simulink model "supplemental_network"  (R2023b)
settings: Solver=ode3  StartTime=0.0  StopTime=sup_cfg.stop  FixedStep=sup_cfg.electricalStep  RelTol=1e-6
InitFcn:
  | Rf=0.05;Lf=2e-3;Cf=50e-6;fn=50;w0=2*fn*pi;
  | UB=3e3;SB=1e6;IB=SB/(sqrt(3)*UB);
  | Xf=Lf*w0;Z=sqrt((Rf^2+Xf^2));
  | J=3;D=2e4/w0*0;kf=0.9e4/w0;
  | K=230*380/Xf;
  | P=10;I=12e3;
  | Jw=8e4;
  | Pi=1;Pp=0;P2 =1000;
  | U5=30;
  | U7=15;
undefined symbols (not defined in the file): sup_cfg
libraries: slpidlib x5, spsThreePhaseSeriesRLCBranchLib x4, spsControlledVoltageSourceLib x4, spsControlledCurrentSourceLib x3, spsThreePhaseBreakerLib x3, spsabctodq0Lib x3, spsThreePhaseVIMeasurementLib x3, spsGroundLib x2, spsThreePhaseSeriesRLCLoadLib x2, spsUniversalBridgeLib x1, spsPWMGenerator2LevelLib x1, spsdq0toabcLib x1
settings Model: Creator=lenovo  LastModifiedBy=yangweilin
settings SolverCC: ZeroCrossAlgorithm=Adaptive  AlgebraicLoopSolver=TrustRegion
settings DataIOCC: SaveFormat=StructureWithTime  SignalLogging=off
settings OptimizationCC: DefaultParameterBehavior=Inlined  EnhancedBackFolding=on  PassReuseOutputArgsAs=Individual arguments  ZeroExternalMemoryAtStartup=off  ZeroInternalMemoryAtStartup=off  AccelVerboseBuild=on  OptimizeBlockOrder=speed  DifferentSizesBufferReuse=on  OptimizationCustomize=off  EfficientTunableParamExpr=on
settings DebuggingCC: IgnoredZcDiagnostic=none  ParameterTunabilityLossMsg=error  UnconnectedInputMsg=warning  UnconnectedOutputMsg=warning  UnconnectedLineMsg=warning  ArithmeticOperatorsInVariantConditions=warning
settings ModelReferenceCC: EnableRefExpFcnMdlSchedulingChecks=on
settings SFSimCC: MATLABDynamicMemAlloc=off  CustomCodeUndefinedFunction=UseInterfaceOnly
settings RTWCC: Description=Embedded Coder  SystemTargetFile=ert.tlc  TemplateMakefile=ert_default_tmf
settings CodeAppCC: ForceParamTrailComments=on  IgnoreCustomStorageClasses=off  OperatorAnnotations=on  SimulinkDataObjDesc=on  SFDataObjDesc=on  InsertBlockDesc=on
settings ERTTargetCC: TargetLangStandard=C99 (ISO)  GenerateSampleERTMain=on  InlinedParameterPlacement=NonHierarchical  ERTCustomFileTemplate=example_file_process.tlc

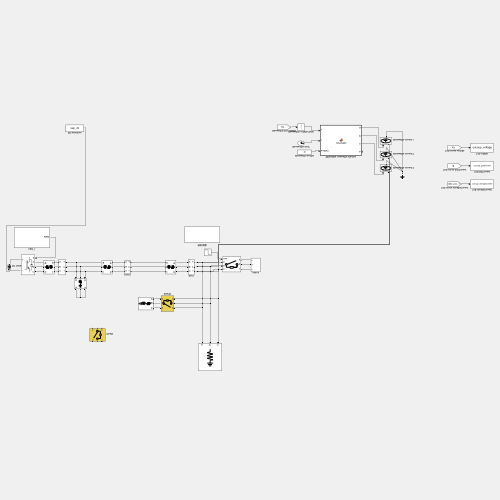
[thumbnail: Simulink's stored preview of the top-level diagram]
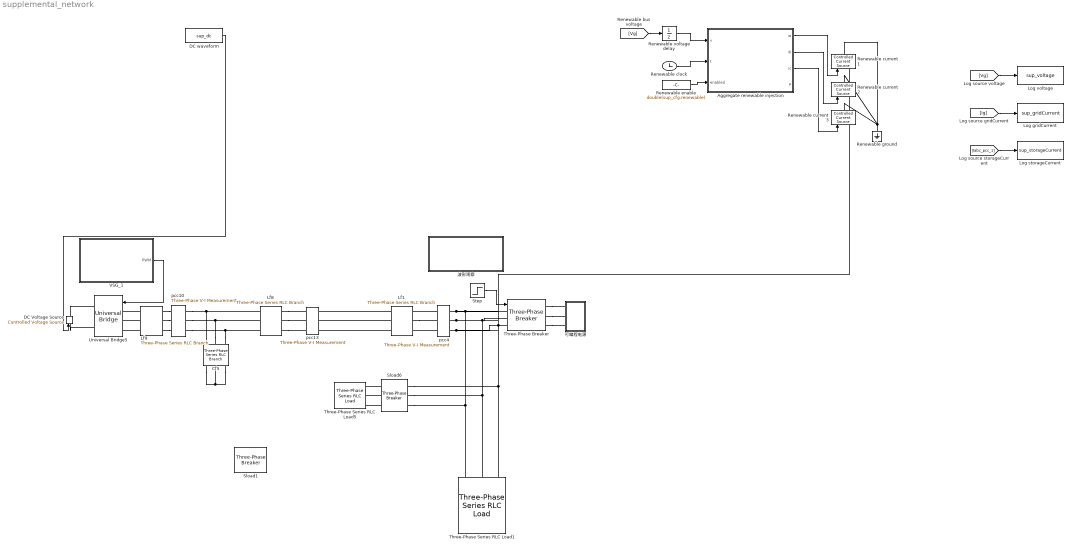
== system supplemental_network ==
  " Lf1" : spsThreePhaseSeriesRLCBranchLib/Three-Phase Series RLC Branch  LConnTagsString=A|B|C  RConnTagsString=A|B|C  BranchType=RL  Resistance=0.1  Inductance=0.0002  Capacitance=0  Measurements=None
  " Lf8" : spsThreePhaseSeriesRLCBranchLib/Three-Phase Series RLC Branch  LConnTagsString=A|B|C  RConnTagsString=A|B|C  BranchType=RL  Resistance=0.02  Inductance=0.004  Capacitance=0  Measurements=None
  " Lf9" : spsThreePhaseSeriesRLCBranchLib/Three-Phase Series RLC Branch  LConnTagsString=A|B|C  RConnTagsString=A|B|C  BranchType=RL  Resistance=0.1  Inductance=0.005  Capacitance=0  Measurements=None
  Aggregate renewable injection : MATLAB Function  TreatAsAtomicUnit=on
  Cf5 : spsThreePhaseSeriesRLCBranchLib/Three-Phase Series RLC Branch  LConnTagsString=A|B|C  RConnTagsString=A|B|C  BranchType=RC  Resistance=0.5  Inductance=4e-3  Capacitance=3e-5  Measurements=None
  DC Voltage Source : spsControlledVoltageSourceLib/Controlled Voltage Source  Initialize=on  Source_Type=DC  Amplitude=800  Phase=0  Frequency=0  Measurements=None
  DC waveform : FromWorkspace  VariableName=sup_dc  Interpolate=off  OutputAfterFinalValue=Holding final value
  Log gridCurrent : ToWorkspace  VariableName=sup_gridCurrent  SaveFormat=Structure With Time  SampleTime=sup_cfg.Ts
  Log storageCurrent : ToWorkspace  VariableName=sup_storageCurrent  SaveFormat=Structure With Time  SampleTime=sup_cfg.Ts
  Log voltage : ToWorkspace  VariableName=sup_voltage  SaveFormat=Structure With Time  SampleTime=sup_cfg.Ts
  Renewable clock : Clock
  Renewable current 1 : spsControlledCurrentSourceLib/Controlled Current Source  Initialize=on  Source_Type=DC  Amplitude=0  Phase=0  Frequency=0  Measurements=None
  Renewable current 2 : spsControlledCurrentSourceLib/Controlled Current Source  Initialize=on  Source_Type=DC  Amplitude=0  Phase=0  Frequency=0  Measurements=None
  Renewable current 3 : spsControlledCurrentSourceLib/Controlled Current Source  Initialize=on  Source_Type=DC  Amplitude=0  Phase=0  Frequency=0  Measurements=None
  Renewable enable : Constant  Value=double(sup_cfg.renewable)
  Renewable ground : spsGroundLib/Ground  LConnTagsString=a
  Renewable voltage delay : UnitDelay  InitialCondition=[0;0;0]  SampleTime=sup_cfg.electricalStep  HasFrameUpgradeWarning=on
  Sload1 : spsThreePhaseBreakerLib/Three-Phase Breaker  InitialState=open  SwitchA=on  SwitchB=on  SwitchC=on  SwitchTimes=[1.0]  External=off  BreakerResistance=0.0001  SnubberResistance=1e6  SnubberCapacitance=inf  Measurements=None
  Sload6 : spsThreePhaseBreakerLib/Three-Phase Breaker  InitialState=open  SwitchA=on  SwitchB=on  SwitchC=on  SwitchTimes=[1.2]  External=off  BreakerResistance=0.0001  SnubberResistance=1e6  SnubberCapacitance=inf  Measurements=None
  Step : Step  Before=1  After=0  SampleTime=0
  Three-Phase Series RLC Load1 : spsThreePhaseSeriesRLCLoadLib/Three-Phase Series RLC Load  LConnTagsString=A|B|C  Configuration=Y (grounded)  NominalVoltage=380  Vabc=[1e3 1e3 1e3]  Vabcp=[1e3 1e3 1e3]  NominalFrequency=50  UnbalancedPower=off  ActivePower=15e3  InductivePower=0  CapacitivePower=0  Pabc=[10e3 9e3 11e3]  QLabc=[100 90 110]  QCabc=[100 90 110]  Pabcp=[10e3 9e3 11e3]  QLabcp=[100 90 110]  QCabcp=[100 90 110]  Measurements=None  LoadType=constant Z
  Three-Phase Series RLC Load5 : spsThreePhaseSeriesRLCLoadLib/Three-Phase Series RLC Load  LConnTagsString=A|B|C  Configuration=Y (grounded)  NominalVoltage=380  Vabc=[1e3 1e3 1e3]  Vabcp=[1e3 1e3 1e3]  NominalFrequency=50  UnbalancedPower=off  ActivePower=15e3  InductivePower=6e3  CapacitivePower=0  Pabc=[10e3 9e3 11e3]  QLabc=[100 90 110]  QCabc=[100 90 110]  Pabcp=[10e3 9e3 11e3]  QLabcp=[100 90 110]  QCabcp=[100 90 110]  Measurements=None  LoadType=constant Z
  Three-Phase Breaker : spsThreePhaseBreakerLib/Three-Phase Breaker  InitialState=open  SwitchA=on  SwitchB=on  SwitchC=on  SwitchTimes="[1/60  5/60]"  External=on  BreakerResistance=0.01  SnubberResistance=1e6  SnubberCapacitance=inf  Measurements=None
  Universal Bridge5 : spsUniversalBridgeLib/Universal Bridge  Arms=3  SnubberResistance=1e5  SnubberCapacitance=inf  Device=IGBT / Diodes  Ron=1e-5  Lon=0  ForwardVoltages=[0.05 0.05]  ForwardVoltage=0  GTOparameters=[ 10e-6 , 20e-6 ]  IGBTparameters=[ 1e-6 , 2e-6 ]  Measurements=None  Measurements_2=None  converterType=Rectifier
  VSG_1 : Subsystem
  pcc10 : spsThreePhaseVIMeasurementLib/Three-Phase V-I Measurement  VoltageMeasurement=phase-to-ground  SetLabelV=on  LabelV=Vo_1  Vpu=off  VpuLL=off  CurrentMeasurement=yes  SetLabelI=on  LabelI=IL_1  Ipu=off  Pbase=1e6  Vbase=6.6e3/sqrt(3)  OutputType=Magnitude  PhasorSimulation=off  PSBequivalent=0
  pcc13 : spsThreePhaseVIMeasurementLib/Three-Phase V-I Measurement  VoltageMeasurement=phase-to-ground  SetLabelV=on  LabelV=Vabc_pcc_1  Vpu=off  VpuLL=off  CurrentMeasurement=yes  SetLabelI=on  LabelI=Iabc_pcc_1  Ipu=off  Pbase=1e6  Vbase=6.6e3/sqrt(3)  OutputType=Magnitude  PhasorSimulation=off  PSBequivalent=0
  pcc4 : spsThreePhaseVIMeasurementLib/Three-Phase V-I Measurement  VoltageMeasurement=phase-to-ground  SetLabelV=on  LabelV=Vg  Vpu=off  VpuLL=off  CurrentMeasurement=yes  SetLabelI=on  LabelI=Ig  Ipu=off  Pbase=1e6  Vbase=6.6e3/sqrt(3)  OutputType=Magnitude  PhasorSimulation=off  PSBequivalent=0
  可编程电源 : Subsystem
  波形观察 : Subsystem
  wires:
  VSG_1/1(PWM) -> Universal Bridge5/1
  Step/1 -> Three-Phase Breaker/1
  DC waveform/1 -> DC Voltage Source/1
  [Vg] -> Renewable voltage delay/1
  Renewable voltage delay/1 -> Aggregate renewable injection/1(v)
  Renewable clock/1 -> Aggregate renewable injection/2(t)
  Renewable enable/1 -> Aggregate renewable injection/3(enabled)
  Aggregate renewable injection/1(ia) -> Renewable current 1/1
  Aggregate renewable injection/2(ib) -> Renewable current 2/1
  Aggregate renewable injection/3(ic) -> Renewable current 3/1
  [Vg] -> Log voltage/1
  [Ig] -> Log gridCurrent/1
  [Iabc_pcc_1] -> Log storageCurrent/1
  connections:
  Cf5/RConn2 -- Cf5/RConn3 -- Cf5/RConn1
  " Lf9"/LConn3 -- Universal Bridge5/LConn3
  " Lf9"/LConn1 -- Universal Bridge5/LConn1
  " Lf9"/LConn2 -- Universal Bridge5/LConn2
  " Lf8"/RConn1 -- pcc10/RConn1 -- Cf5/LConn1
  Cf5/LConn3 -- pcc10/RConn3 -- " Lf8"/RConn3
  Cf5/LConn2 -- pcc10/RConn2 -- " Lf8"/RConn2
  " Lf1"/LConn2 -- pcc4/LConn2
  pcc4/LConn3 -- " Lf1"/LConn3
  pcc4/LConn1 -- " Lf1"/LConn1
  " Lf1"/RConn1 -- pcc13/RConn1
  " Lf1"/RConn2 -- pcc13/RConn2
  " Lf1"/RConn3 -- pcc13/RConn3
  " Lf8"/LConn1 -- pcc13/LConn1
  " Lf8"/LConn2 -- pcc13/LConn2
  " Lf8"/LConn3 -- pcc13/LConn3
  DC Voltage Source/RConn1 -- Universal Bridge5/RConn1
  DC Voltage Source/LConn1 -- Universal Bridge5/RConn2
  " Lf9"/RConn1 -- pcc10/LConn1
  " Lf9"/RConn2 -- pcc10/LConn2
  " Lf9"/RConn3 -- pcc10/LConn3
  Three-Phase Breaker/RConn1 -- 可编程电源/RConn1
  Three-Phase Breaker/RConn2 -- 可编程电源/RConn2
  Three-Phase Breaker/RConn3 -- 可编程电源/RConn3
  Sload6/LConn3 -- Three-Phase Series RLC Load5/LConn1
  Sload6/LConn2 -- Three-Phase Series RLC Load5/LConn2
  Sload6/LConn1 -- Three-Phase Series RLC Load5/LConn3
  Three-Phase Breaker/LConn1 -- Three-Phase Series RLC Load1/LConn1 -- Sload6/RConn1 -- pcc4/RConn1 -- Renewable current 1/LConn1
  pcc4/RConn2 -- Renewable current 2/LConn1 -- Three-Phase Series RLC Load1/LConn2 -- Sload6/RConn2 -- Three-Phase Breaker/LConn2
  Three-Phase Breaker/LConn3 -- Sload6/RConn3 -- Three-Phase Series RLC Load1/LConn3 -- pcc4/RConn3 -- Renewable current 3/LConn1
  Renewable current 1/RConn1 -- Renewable current 2/RConn1 -- Renewable ground/LConn1 -- Renewable current 3/RConn1

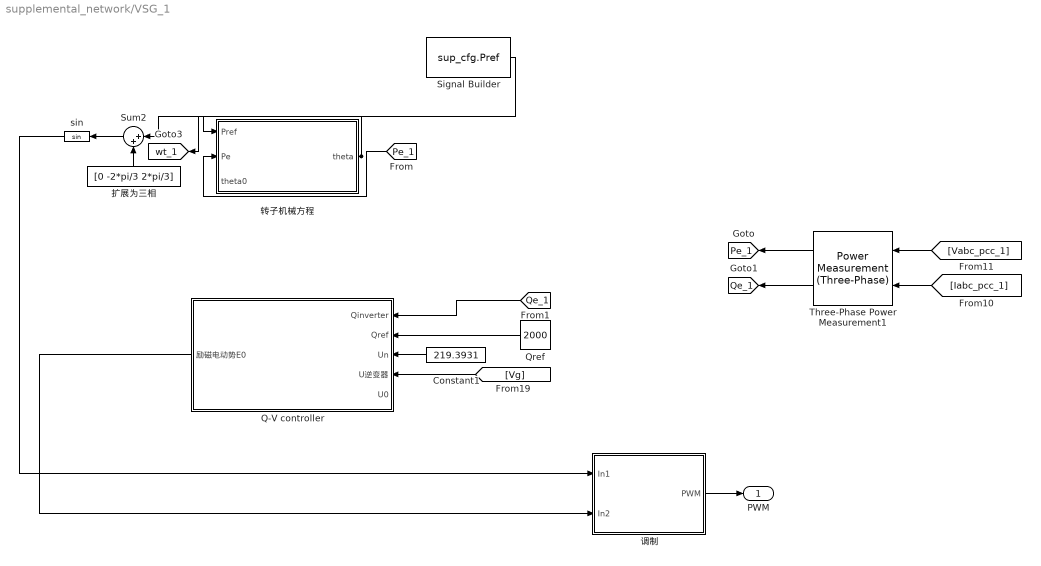
== system supplemental_network/VSG_1 ==
  " 调制" : Subsystem
  Constant1 : Constant  Value=219.3931
  Q-V controller : Subsystem
  Qref : Constant  Value=2000
  Signal Builder : Constant  Value=sup_cfg.Pref
  Sum2 : Sum  Inputs=|++
  Three-Phase Power Measurement1 : eePowerMeasurement/Power Measurement (Three-Phase)  LabelModeActiveChoice=Continuous  F=50  K=[1]  Seq=Positive  Ts=0
  sin : Trigonometry
  扩展为三相 : Constant  Value=[0 -2*pi/3 2*pi/3]
  转子机械方程 : Subsystem
  PWM : Outport
  tag scope: Pe_1=global, Qe_1=global, wt_1=global
  wires:
  扩展为三相/1 -> Sum2/2
  Three-Phase Power Measurement1/1 -> [Pe_1]
  [Iabc_pcc_1] -> Three-Phase Power Measurement1/2
  Qref/1 -> Q-V controller/2(Qref)
  [Vg] -> Q-V controller/4(U逆变器)
  [Vabc_pcc_1] -> Three-Phase Power Measurement1/1
  Three-Phase Power Measurement1/2 -> [Qe_1]
  Constant1/1 -> Q-V controller/3(Un)
  Sum2/1 -> sin/1
  sin/1 -> " 调制"/1(In1)
  Q-V controller/1(励磁电动势E0) -> " 调制"/2(In2)
  " 调制"/1(PWM) -> PWM/1
  [Qe_1] -> Q-V controller/1(Qinverter)
  [Pe_1] -> 转子机械方程/2(Pe)
  转子机械方程/1(theta) -> Sum2/1, [wt_1]
  Signal Builder/1 -> 转子机械方程/1(Pref)

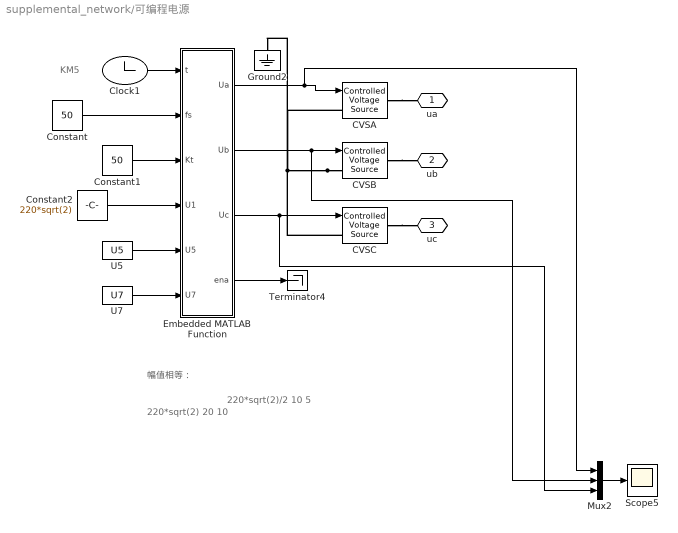
== system supplemental_network/可编程电源 ==
  note: KM5
  note: 幅值相等：
  note: 220*sqrt(2)
      | 20
      | 10
  note: 220*sqrt(2)/2
      | 10
      | 5
  CVSA : spsControlledVoltageSourceLib/Controlled Voltage Source  Initialize=on  Source_Type=AC  Amplitude=0  Phase=0  Frequency=0  Measurements=None
  CVSB : spsControlledVoltageSourceLib/Controlled Voltage Source  Initialize=on  Source_Type=AC  Amplitude=0  Phase=0  Frequency=0  Measurements=None
  CVSC : spsControlledVoltageSourceLib/Controlled Voltage Source  Initialize=on  Source_Type=AC  Amplitude=0  Phase=0  Frequency=0  Measurements=None
  Clock1 : Clock
  Constant : Constant  Value=50
  Constant1 : Constant  Value=50
  Constant2 : Constant  Value=220*sqrt(2)
  Embedded MATLAB Function : MATLAB Function  TreatAsAtomicUnit=on
  Ground2 : spsGroundLib/Ground  LConnTagsString=a
  Mux2 : Mux  Inputs=3
  Scope5 : Scope
  Terminator4 : Terminator
  U5 : Constant  Value=U5
  U7 : Constant  Value=U7
  ua : PMIOPort  Side=Right
  ub : PMIOPort  Port=2  Side=Right
  uc : PMIOPort  Port=3  Side=Right
  wires:
  Clock1/1 -> Embedded MATLAB Function/1(t)
  U5/1 -> Embedded MATLAB Function/5(U5)
  Embedded MATLAB Function/3(Uc) -> Mux2/3, CVSC/1
  U7/1 -> Embedded MATLAB Function/6(U7)
  Embedded MATLAB Function/4(ena) -> Terminator4/1
  Constant1/1 -> Embedded MATLAB Function/3(Kt)
  Constant/1 -> Embedded MATLAB Function/2(fs)
  Embedded MATLAB Function/2(Ub) -> Mux2/2, CVSB/1
  Mux2/1 -> Scope5/1
  Embedded MATLAB Function/1(Ua) -> Mux2/1, CVSA/1
  Constant2/1 -> Embedded MATLAB Function/4(U1)
  connections:
  CVSC/RConn1 -- uc/RConn1
  CVSB/RConn1 -- ub/RConn1
  CVSA/RConn1 -- ua/RConn1
  CVSB/LConn1 -- Ground2/LConn1 -- CVSA/LConn1 -- CVSC/LConn1

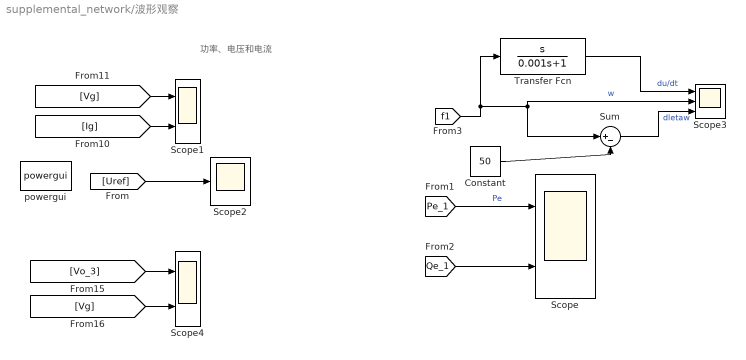
== system supplemental_network/波形观察 ==
  note: 功率、电压和电流
  Constant : Constant  Value=50
  Scope : Scope  NumInputPorts=2
  Scope1 : Scope  NumInputPorts=2
  Scope2 : Scope
  Scope3 : Scope  NumInputPorts=3
  Scope4 : Scope  NumInputPorts=2
  Sum : Sum  Inputs=|+-
  Transfer Fcn : TransferFcn  Numerator=[1 0]  Denominator=[0.001 1]
  powergui : spspowerguiLib/powergui  Priority=1  SimulationMode=Discrete  SampleTime=sup_cfg.electricalStep  frequency=60  Iterations=50  frequencyindice=0  Pbase=100e6  ErrMax=1e-4  UnitsV=kV  UnitsW=MW  buscounter=0  FunctionMessages=off  echomessages=off  EnableUseOfTLC=off  CurrentSourceSwitches=off  DisableSnubberDevices=off  DisableRonSwitches=off  DisableVfSwitches=off  DisplayEquations=off  AutomaticDiscreteSolvers=off  SolverType=Tustin/Backward Euler (TBE)  Interpol=off  ExternalGateDelay=off  methode=off  Ts=100  x0status=blocks  SPID=on  SwTol=0  HookPort=off  NonlinearTolerance=1e-4  nMaxIteration=100  ContinueOnMaxIteration=off  RestoreLinks=warning  ResistiveCurrentMeasurement=off  Frange=[0:2:500]  Ylog=off  Xlog=on  ShowGrid=off  save=off  variable=ZData  structure=logsout  ZoomFFT=off  StartTime=0.5  cycles=10  DisplayStyle=1  fundamental=50  FreqAxis=off  MaxFrequency=1000  frequencyindicesteady=1  RmsSteady=1  display=off
  wires:
  [Vg] -> Scope1/1
  [Qe_1] -> Scope/2
  [Pe_1] -> Scope/1  "Pe"
  [Ig] -> Scope1/2
  [Uref] -> Scope2/1
  [f1] -> Sum/1, Scope3/2, Transfer Fcn/1  "w"
  [Vo_3] -> Scope4/1
  [Vg] -> Scope4/2
  Transfer Fcn/1 -> Scope3/1  "du/dt"
  Constant/1 -> Sum/2
  Sum/1 -> Scope3/3  "dletaw"

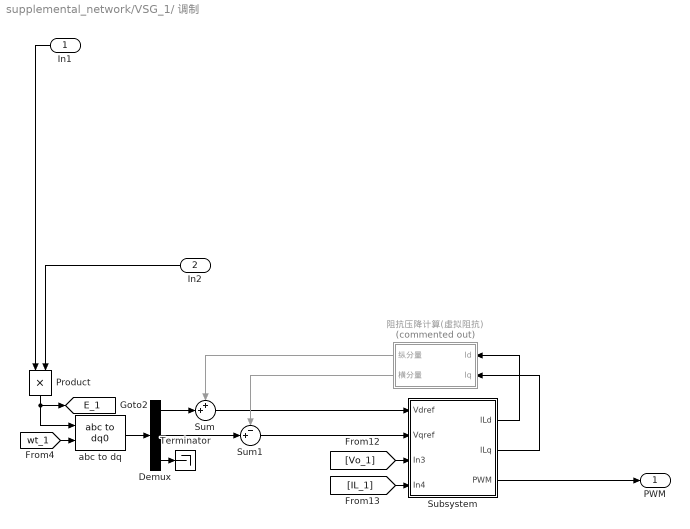
== system supplemental_network/VSG_1/ 调制 ==
  In1 : Inport
  In2 : Inport  Port=2
  Demux : Demux  Outputs=3
  Product : Product
  Subsystem : Subsystem
  Sum : Sum  Inputs=++|
  Sum1 : Sum  Inputs=-+|
  Terminator : Terminator
  abc to dq : spsabctodq0Lib/abc to dq0  Alignment=90 degrees behind phase A axis
  阻抗压降计算(虚拟阻抗) : Subsystem  Commented=on
  PWM : Outport
  tag scope: E_1=global
  wires:
  [Vo_1] -> Subsystem/3(In3)
  Demux/2 -> Sum1/2
  Sum/1 -> Subsystem/1(Vdref)
  [IL_1] -> Subsystem/4(In4)
  abc to dq/1 -> Demux/1
  Subsystem/1(ILd) -> 阻抗压降计算(虚拟阻抗)/1(Id)
  Demux/1 -> Sum/2
  阻抗压降计算(虚拟阻抗)/1(纵分量) -> Sum/1
  Demux/3 -> Terminator/1
  Sum1/1 -> Subsystem/2(Vqref)
  Product/1 -> [E_1], abc to dq/1
  Subsystem/2(ILq) -> 阻抗压降计算(虚拟阻抗)/2(Iq)
  阻抗压降计算(虚拟阻抗)/2(横分量) -> Sum1/1
  Subsystem/3(PWM) -> PWM/1
  [wt_1] -> abc to dq/2
  In1/1 -> Product/1
  In2/1 -> Product/2

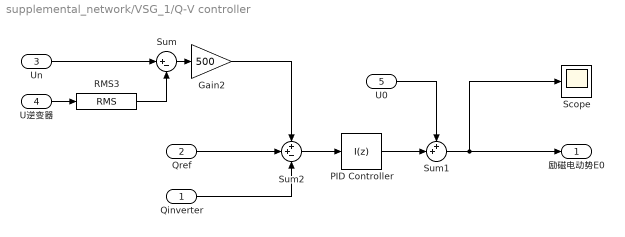
== system supplemental_network/VSG_1/Q-V controller ==
  Qinverter : Inport
  Qref : Inport  Port=2
  Un : Inport  Port=3
  U逆变器 : Inport  Port=4
  U0 : Inport  Port=5
  Gain2 : Gain  Gain=500
  PID Controller : slpidlib/PID Controller  Controller=I  Form=Parallel  TimeDomain=Discrete-time  UseExternalTs=off  SampleTime=-1  IntegratorMethod=Forward Euler  FilterMethod=Forward Euler  ControllerParametersSource=internal  P=0.0000001  I=1.1547e-5*5  UseKiTs=off  D=0  N=100  UseFilter=on  TunerSelectOption=Transfer Function Based (PID Tuner App)  InitialConditionSource=internal  InitialConditionForIntegrator=0  InitialConditionForFilter=0  DifferentiatorICPrevScaledInput=0  ExternalReset=none  TrackingMode=off  Kt=1  LimitOutput=off  SatLimitsSource=internal  UpperSaturationLimit=inf  LowerSaturationLimit=-inf  LinearizeAsGain=on  AntiWindupMode=none  Kb=1  LimitIntegrator=off  UpperIntegratorSaturationLimit=inf  LowerIntegratorSaturationLimit=-inf  POutMin=[]  POutMax=[]  IOutMin=[]  IOutMax=[]  DOutMin=[]  DOutMax=[]  NOutMin=[]  NOutMax=[]  SumOutMin=[]  SumOutMax=[]  SaturationOutMin=[]  SaturationOutMax=[]  PParamMin=[]  PParamMax=[]  IParamMin=[]  IParamMax=[]  DParamMin=[]  DParamMax=[]  NParamMin=[]  NParamMax=[]  KbParamMin=[]  KbParamMax=[]  KtParamMin=[]  KtParamMax=[]  KbOutMin=[]  KbOutMax=[]  KtOutMin=[]  KtOutMax=[]  IntegratorOutMin=[]  IntegratorOutMax=[]  FilterOutMin=[]  FilterOutMax=[]  SumI1OutMin=[]  SumI1OutMax=[]  SumI2OutMin=[]  SumI2OutMax=[]  SumI3OutMin=[]  SumI3OutMax=[]  SumI4OutMin=[]  SumI4OutMax=[]  SumDOutMin=[]  SumDOutMax=[]  DifferentiatorOutMin=[]  DifferentiatorOutMax=[]  FilterDiffOutCoefMin=[]  FilterDiffOutCoefMax=[]  ReciprocalOutMin=[]  ReciprocalOutMax=[]  SumDenOutMin=[]  SumDenOutMax=[]  SumNumOutMin=[]  SumNumOutMax=[]  DivideOutMin=[]  DivideOutMax=[]  UdiffTsProdOutMin=[]  UdiffTsProdOutMax=[]  NTsProdOutMin=[]  NTsProdOutMax=[]  UintegralTsProdOutMin=[]  UintegralTsProdOutMax=[]  UngainTsProdOutMin=[]  UngainTsProdOutMax=[]  ClampingZeroOutDataTypeStr=Inherit: Inherit via back propagation  ClampingZeroOutMin=[]  ClampingZeroOutMax=[]  FilterDenConstantOutDataTypeStr=Inherit: Inherit via back propagation  FilterDenConstantOutMin=[]  FilterDenConstantOutMax=[]  PCopyOutDataTypeStr=Inherit: Inherit via back propagation  PCopyOutMin=[]  PCopyOutMax=[]  NCopyOutDataTypeStr=Inherit: Inherit via back propagation  NCopyOutMin=[]  NCopyOutMax=[]  IntegratorContinuousStateAttributes=''  IntegratorStateMustResolveToSignalObject=off  IntegratorRTWStateStorageClass=Auto  FilterContinuousStateAttributes=''  FilterStateMustResolveToSignalObject=off  FilterRTWStateStorageClass=Auto  ParallelPVariant=Disabled  IdealPVariant=Disabled  IVariant=InternalParameters  DVariant=Disabled  IntegratorVariant=Discrete  SatVariant=Disabled  AWVariant=Passthrough  PCopyVariant=Disabled  TRVariant=Disabled  FdbkBlocksVariant=Forward  IdealPFdbkVariant=Disabled  SatFdbkVariant=Disabled  DerivativeFilterVariant=Disabled  NVariant=Disabled  NCopyVariant=Disabled_SignalSpec  FilterICVariant=Disabled  IntegratorICVariant=InternalICs  ExternalResetVariant=Disabled  TRSumVariant=Passthrough  SumFdbkVariant=Disabled  SumVariant=Passthrough_I  TsampFilterVariant=InternalTs  TsampNgainVariant=Passthrough  TsampIntegralVariant=Disabled_SignalSpec  ExternalSaturationOutDataTypeStr=Inherit: Same as second input
  RMS3 : dspstat3/RMS  run=off  directionMode=Each column  dimension=1  InputProcessing=Columns as channels (frame based)  reset_popup=None
  Scope : Scope
  Sum : Sum  Inputs=|+-
  Sum1 : Sum  Inputs=++|
  Sum2 : Sum  Inputs=++-
  励磁电动势E0 : Outport
  wires:
  Qinverter/1 -> Sum2/3
  Qref/1 -> Sum2/2
  Un/1 -> Sum/1
  U逆变器/1 -> RMS3/1
  Gain2/1 -> Sum2/1
  Sum/1 -> Gain2/1
  RMS3/1 -> Sum/2
  Sum2/1 -> PID Controller/1
  U0/1 -> Sum1/1
  Sum1/1 -> 励磁电动势E0/1, Scope/1
  PID Controller/1 -> Sum1/2

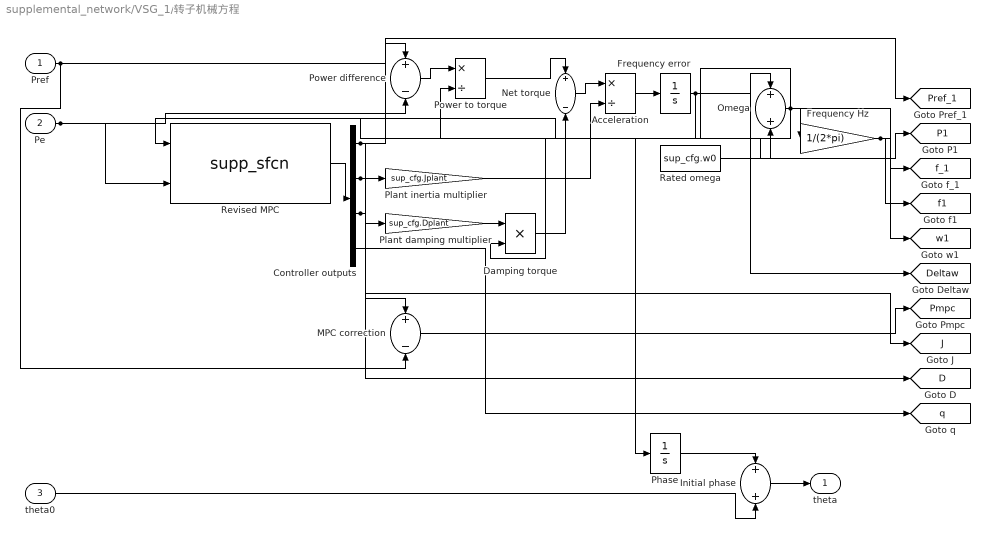
== system supplemental_network/VSG_1/转子机械方程 ==
  Pref : Inport
  Pe : Inport  Port=2
  theta0 : Inport  Port=3
  Acceleration : Product  Inputs=*/
  Controller outputs : Demux
  Damping torque : Product  Inputs=**
  Frequency Hz : Gain  Gain=1/(2*pi)
  Frequency error : Integrator
  Initial phase : Sum
  MPC correction : Sum  Inputs=+-
  Net torque : Sum  Inputs=+-
  Omega : Sum
  Phase : Integrator
  Plant damping multiplier : Gain  Gain=sup_cfg.Dplant
  Plant inertia multiplier : Gain  Gain=sup_cfg.Jplant
  Power difference : Sum  Inputs=+-
  Power to torque : Product  Inputs=*/
  Rated omega : Constant  Value=sup_cfg.w0
  Revised MPC : M-S-Function  FunctionName=supp_sfcn  Parameters=sup_cfg
  theta : Outport
  tag scope: D=global, Deltaw=global, J=global, P1=global, Pmpc=global, Pref_1=global, f1=global, f_1=global, q=global, w1=global
  wires:
  Pe/1 -> Revised MPC/2, Power difference/2, [P1]
  Omega/1 -> Revised MPC/1, Power to torque/2, Frequency Hz/1, Phase/1, [w1]
  Revised MPC/1 -> Controller outputs/1
  Controller outputs/1 -> Power difference/1, MPC correction/1
  Power difference/1 -> Power to torque/1
  Controller outputs/2 -> Plant inertia multiplier/1, [J]
  Controller outputs/3 -> Plant damping multiplier/1, [D]
  Plant damping multiplier/1 -> Damping torque/1
  Frequency error/1 -> Damping torque/2, Omega/1, [Deltaw]
  Power to torque/1 -> Net torque/1
  Damping torque/1 -> Net torque/2
  Net torque/1 -> Acceleration/1
  Plant inertia multiplier/1 -> Acceleration/2
  Acceleration/1 -> Frequency error/1
  Rated omega/1 -> Omega/2
  Phase/1 -> Initial phase/1
  theta0/1 -> Initial phase/2
  Initial phase/1 -> theta/1
  Pref/1 -> MPC correction/2, [Pref_1]
  Frequency Hz/1 -> [f_1], [f1]
  MPC correction/1 -> [Pmpc]
  Controller outputs/4 -> [q]

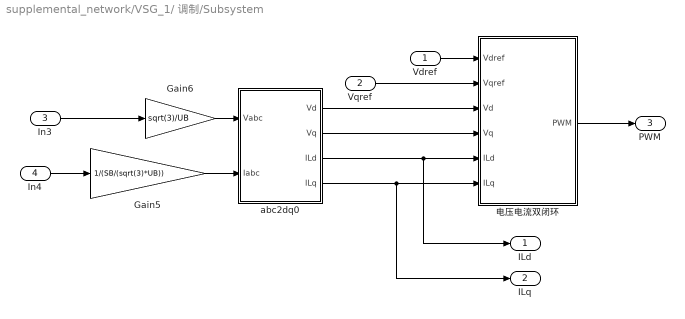
== system supplemental_network/VSG_1/ 调制/Subsystem ==
  Vdref : Inport
  Vqref : Inport  Port=2
  In3 : Inport  Port=3
  In4 : Inport  Port=4
  Gain5 : Gain  Gain=1/(SB/(sqrt(3)*UB))
  Gain6 : Gain  Gain=sqrt(3)/UB
  abc2dq0 : Subsystem
  电压电流双闭环 : Subsystem
  ILd : Outport
  ILq : Outport  Port=2
  PWM : Outport  Port=3
  wires:
  Vqref/1 -> 电压电流双闭环/2(Vqref)
  In4/1 -> Gain5/1
  abc2dq0/1(Vd) -> 电压电流双闭环/3(Vd)
  abc2dq0/2(Vq) -> 电压电流双闭环/4(Vq)
  abc2dq0/3(ILd) -> 电压电流双闭环/5(ILd), ILd/1
  Gain5/1 -> abc2dq0/2(Iabc)
  Gain6/1 -> abc2dq0/1(Vabc)
  abc2dq0/4(ILq) -> 电压电流双闭环/6(ILq), ILq/1
  电压电流双闭环/1(PWM) -> PWM/1
  Vdref/1 -> 电压电流双闭环/1(Vdref)
  In3/1 -> Gain6/1

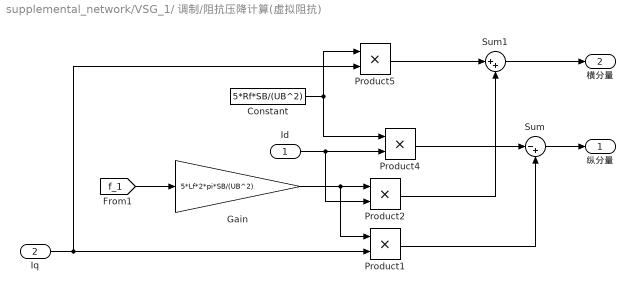
== system supplemental_network/VSG_1/ 调制/阻抗压降计算(虚拟阻抗) ==
  Id : Inport
  Iq : Inport  Port=2
  Constant : Constant  Value=5*Rf*SB/(UB^2)
  Gain : Gain  Gain=5*Lf*2*pi*SB/(UB^2)
  Product{1..2,4..5} (4 alike) : Product
  Sum : Sum  Inputs=|-+
  Sum1 : Sum  Inputs=|++
  纵分量 : Outport
  横分量 : Outport  Port=2
  wires:
  Product2/1 -> Sum1/2
  Sum1/1 -> 横分量/1
  Product5/1 -> Sum1/1
  Sum/1 -> 纵分量/1
  Product1/1 -> Sum/2
  Product4/1 -> Sum/1
  Gain/1 -> Product1/1, Product2/1
  Iq/1 -> Product5/2, Product1/2
  [f_1] -> Gain/1
  Constant/1 -> Product5/1, Product4/1
  Id/1 -> Product2/2, Product4/2

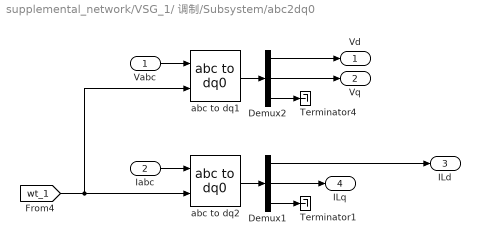
== system supplemental_network/VSG_1/ 调制/Subsystem/abc2dq0 ==
  Vabc : Inport
  Iabc : Inport  Port=2
  Demux1 : Demux  Outputs=3
      settings: DisplayOption=none
  Demux2 : Demux  Outputs=3
      settings: DisplayOption=none
  Terminator1 : Terminator
  Terminator4 : Terminator
  abc to dq1 : spsabctodq0Lib/abc to dq0  Alignment=90 degrees behind phase A axis
  abc to dq2 : spsabctodq0Lib/abc to dq0  Alignment=90 degrees behind phase A axis
  Vd : Outport
  Vq : Outport  Port=2
  ILd : Outport  Port=3
  ILq : Outport  Port=4
  wires:
  [wt_1] -> abc to dq2/2, abc to dq1/2
  Vabc/1 -> abc to dq1/1
  abc to dq1/1 -> Demux2/1
  Iabc/1 -> abc to dq2/1
  Demux2/3 -> Terminator4/1
  abc to dq2/1 -> Demux1/1
  Demux1/3 -> Terminator1/1
  Demux1/2 -> ILq/1
  Demux2/1 -> Vd/1
  Demux1/1 -> ILd/1
  Demux2/2 -> Vq/1

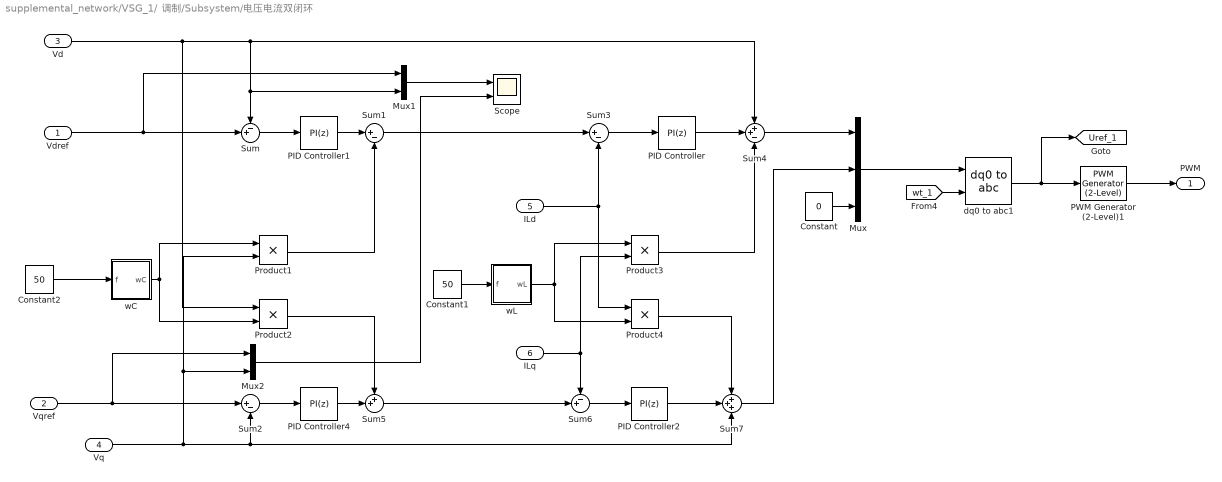
== system supplemental_network/VSG_1/ 调制/Subsystem/电压电流双闭环 ==
  Vdref : Inport
  Vqref : Inport  Port=2
  Vd : Inport  Port=3
  Vq : Inport  Port=4
  ILd : Inport  Port=5
  ILq : Inport  Port=6
  Constant : Constant  Value=0
  Constant1 : Constant  Value=50
  Constant2 : Constant  Value=50
  Mux : Mux  Inputs=3
  Mux1 : Mux  Inputs=2
  Mux2 : Mux  Inputs=2
  PID Controller : slpidlib/PID Controller  Controller=PI  Form=Parallel  TimeDomain=Discrete-time  UseExternalTs=off  SampleTime=-1  IntegratorMethod=Forward Euler  FilterMethod=Forward Euler  ControllerParametersSource=internal  P=1  I=10  UseKiTs=off  D=0  N=100  UseFilter=on  TunerSelectOption=Transfer Function Based (PID Tuner App)  InitialConditionSource=internal  InitialConditionForIntegrator=0  InitialConditionForFilter=0  DifferentiatorICPrevScaledInput=0  ExternalReset=none  TrackingMode=off  Kt=1  LimitOutput=off  SatLimitsSource=internal  UpperSaturationLimit=inf  LowerSaturationLimit=-inf  LinearizeAsGain=on  AntiWindupMode=none  Kb=1  LimitIntegrator=off  UpperIntegratorSaturationLimit=inf  LowerIntegratorSaturationLimit=-inf  POutMin=[]  POutMax=[]  IOutMin=[]  IOutMax=[]  DOutMin=[]  DOutMax=[]  NOutMin=[]  NOutMax=[]  SumOutMin=[]  SumOutMax=[]  SaturationOutMin=[]  SaturationOutMax=[]  PParamMin=[]  PParamMax=[]  IParamMin=[]  IParamMax=[]  DParamMin=[]  DParamMax=[]  NParamMin=[]  NParamMax=[]  KbParamMin=[]  KbParamMax=[]  KtParamMin=[]  KtParamMax=[]  KbOutMin=[]  KbOutMax=[]  KtOutMin=[]  KtOutMax=[]  IntegratorOutMin=[]  IntegratorOutMax=[]  FilterOutMin=[]  FilterOutMax=[]  SumI1OutMin=[]  SumI1OutMax=[]  SumI2OutMin=[]  SumI2OutMax=[]  SumI3OutMin=[]  SumI3OutMax=[]  SumI4OutMin=[]  SumI4OutMax=[]  SumDOutMin=[]  SumDOutMax=[]  DifferentiatorOutMin=[]  DifferentiatorOutMax=[]  FilterDiffOutCoefMin=[]  FilterDiffOutCoefMax=[]  ReciprocalOutMin=[]  ReciprocalOutMax=[]  SumDenOutMin=[]  SumDenOutMax=[]  SumNumOutMin=[]  SumNumOutMax=[]  DivideOutMin=[]  DivideOutMax=[]  UdiffTsProdOutMin=[]  UdiffTsProdOutMax=[]  NTsProdOutMin=[]  NTsProdOutMax=[]  UintegralTsProdOutMin=[]  UintegralTsProdOutMax=[]  UngainTsProdOutMin=[]  UngainTsProdOutMax=[]  ClampingZeroOutDataTypeStr=Inherit: Inherit via back propagation  ClampingZeroOutMin=[]  ClampingZeroOutMax=[]  FilterDenConstantOutDataTypeStr=Inherit: Inherit via back propagation  FilterDenConstantOutMin=[]  FilterDenConstantOutMax=[]  PCopyOutDataTypeStr=Inherit: Inherit via back propagation  PCopyOutMin=[]  PCopyOutMax=[]  NCopyOutDataTypeStr=Inherit: Inherit via back propagation  NCopyOutMin=[]  NCopyOutMax=[]  IntegratorContinuousStateAttributes=''  IntegratorStateMustResolveToSignalObject=off  IntegratorRTWStateStorageClass=Auto  FilterContinuousStateAttributes=''  FilterStateMustResolveToSignalObject=off  FilterRTWStateStorageClass=Auto  ParallelPVariant=InternalParameters  IdealPVariant=Disabled  IVariant=InternalParameters  DVariant=Disabled  IntegratorVariant=Discrete  SatVariant=Disabled  AWVariant=Passthrough  PCopyVariant=Disabled  TRVariant=Disabled  FdbkBlocksVariant=Forward  IdealPFdbkVariant=Disabled  SatFdbkVariant=Disabled  DerivativeFilterVariant=Disabled  NVariant=Disabled  NCopyVariant=Disabled_SignalSpec  FilterICVariant=Disabled  IntegratorICVariant=InternalICs  ExternalResetVariant=Disabled  TRSumVariant=Passthrough  SumFdbkVariant=Disabled  SumVariant=Sum_PI  TsampFilterVariant=InternalTs  TsampNgainVariant=Passthrough  TsampIntegralVariant=Disabled_SignalSpec  ExternalSaturationOutDataTypeStr=Inherit: Same as second input
  PID Controller1 : slpidlib/PID Controller  Controller=PI  Form=Parallel  TimeDomain=Discrete-time  UseExternalTs=off  SampleTime=-1  IntegratorMethod=Forward Euler  FilterMethod=Forward Euler  ControllerParametersSource=internal  P=P  I=I  UseKiTs=off  D=30  N=100  UseFilter=on  TunerSelectOption=Transfer Function Based (PID Tuner App)  InitialConditionSource=internal  InitialConditionForIntegrator=0  InitialConditionForFilter=0  DifferentiatorICPrevScaledInput=0  ExternalReset=none  TrackingMode=off  Kt=1  LimitOutput=off  SatLimitsSource=internal  UpperSaturationLimit=inf  LowerSaturationLimit=-inf  LinearizeAsGain=on  AntiWindupMode=none  Kb=1  LimitIntegrator=off  UpperIntegratorSaturationLimit=inf  LowerIntegratorSaturationLimit=-inf  POutMin=[]  POutMax=[]  IOutMin=[]  IOutMax=[]  DOutMin=[]  DOutMax=[]  NOutMin=[]  NOutMax=[]  SumOutMin=[]  SumOutMax=[]  SaturationOutMin=[]  SaturationOutMax=[]  PParamMin=[]  PParamMax=[]  IParamMin=[]  IParamMax=[]  DParamMin=[]  DParamMax=[]  NParamMin=[]  NParamMax=[]  KbParamMin=[]  KbParamMax=[]  KtParamMin=[]  KtParamMax=[]  KbOutMin=[]  KbOutMax=[]  KtOutMin=[]  KtOutMax=[]  IntegratorOutMin=[]  IntegratorOutMax=[]  FilterOutMin=[]  FilterOutMax=[]  SumI1OutMin=[]  SumI1OutMax=[]  SumI2OutMin=[]  SumI2OutMax=[]  SumI3OutMin=[]  SumI3OutMax=[]  SumI4OutMin=[]  SumI4OutMax=[]  SumDOutMin=[]  SumDOutMax=[]  DifferentiatorOutMin=[]  DifferentiatorOutMax=[]  FilterDiffOutCoefMin=[]  FilterDiffOutCoefMax=[]  ReciprocalOutMin=[]  ReciprocalOutMax=[]  SumDenOutMin=[]  SumDenOutMax=[]  SumNumOutMin=[]  SumNumOutMax=[]  DivideOutMin=[]  DivideOutMax=[]  UdiffTsProdOutMin=[]  UdiffTsProdOutMax=[]  NTsProdOutMin=[]  NTsProdOutMax=[]  UintegralTsProdOutMin=[]  UintegralTsProdOutMax=[]  UngainTsProdOutMin=[]  UngainTsProdOutMax=[]  ClampingZeroOutDataTypeStr=Inherit: Inherit via back propagation  ClampingZeroOutMin=[]  ClampingZeroOutMax=[]  FilterDenConstantOutDataTypeStr=Inherit: Inherit via back propagation  FilterDenConstantOutMin=[]  FilterDenConstantOutMax=[]  PCopyOutDataTypeStr=Inherit: Inherit via back propagation  PCopyOutMin=[]  PCopyOutMax=[]  NCopyOutDataTypeStr=Inherit: Inherit via back propagation  NCopyOutMin=[]  NCopyOutMax=[]  IntegratorContinuousStateAttributes=''  IntegratorStateMustResolveToSignalObject=off  IntegratorRTWStateStorageClass=Auto  FilterContinuousStateAttributes=''  FilterStateMustResolveToSignalObject=off  FilterRTWStateStorageClass=Auto  ParallelPVariant=InternalParameters  IdealPVariant=Disabled  IVariant=InternalParameters  DVariant=Disabled  IntegratorVariant=Discrete  SatVariant=Disabled  AWVariant=Passthrough  PCopyVariant=Disabled  TRVariant=Disabled  FdbkBlocksVariant=Forward  IdealPFdbkVariant=Disabled  SatFdbkVariant=Disabled  DerivativeFilterVariant=Disabled  NVariant=Disabled  NCopyVariant=Disabled_SignalSpec  FilterICVariant=Disabled  IntegratorICVariant=InternalICs  ExternalResetVariant=Disabled  TRSumVariant=Passthrough  SumFdbkVariant=Disabled  SumVariant=Sum_PI  TsampFilterVariant=InternalTs  TsampNgainVariant=Passthrough  TsampIntegralVariant=Disabled_SignalSpec  ExternalSaturationOutDataTypeStr=Inherit: Same as second input
  PID Controller2 : slpidlib/PID Controller  Controller=PI  Form=Parallel  TimeDomain=Discrete-time  UseExternalTs=off  SampleTime=-1  IntegratorMethod=Forward Euler  FilterMethod=Forward Euler  ControllerParametersSource=internal  P=1  I=10  UseKiTs=off  D=0  N=100  UseFilter=on  TunerSelectOption=Transfer Function Based (PID Tuner App)  InitialConditionSource=internal  InitialConditionForIntegrator=0  InitialConditionForFilter=0  DifferentiatorICPrevScaledInput=0  ExternalReset=none  TrackingMode=off  Kt=1  LimitOutput=off  SatLimitsSource=internal  UpperSaturationLimit=inf  LowerSaturationLimit=-inf  LinearizeAsGain=on  AntiWindupMode=none  Kb=1  LimitIntegrator=off  UpperIntegratorSaturationLimit=inf  LowerIntegratorSaturationLimit=-inf  POutMin=[]  POutMax=[]  IOutMin=[]  IOutMax=[]  DOutMin=[]  DOutMax=[]  NOutMin=[]  NOutMax=[]  SumOutMin=[]  SumOutMax=[]  SaturationOutMin=[]  SaturationOutMax=[]  PParamMin=[]  PParamMax=[]  IParamMin=[]  IParamMax=[]  DParamMin=[]  DParamMax=[]  NParamMin=[]  NParamMax=[]  KbParamMin=[]  KbParamMax=[]  KtParamMin=[]  KtParamMax=[]  KbOutMin=[]  KbOutMax=[]  KtOutMin=[]  KtOutMax=[]  IntegratorOutMin=[]  IntegratorOutMax=[]  FilterOutMin=[]  FilterOutMax=[]  SumI1OutMin=[]  SumI1OutMax=[]  SumI2OutMin=[]  SumI2OutMax=[]  SumI3OutMin=[]  SumI3OutMax=[]  SumI4OutMin=[]  SumI4OutMax=[]  SumDOutMin=[]  SumDOutMax=[]  DifferentiatorOutMin=[]  DifferentiatorOutMax=[]  FilterDiffOutCoefMin=[]  FilterDiffOutCoefMax=[]  ReciprocalOutMin=[]  ReciprocalOutMax=[]  SumDenOutMin=[]  SumDenOutMax=[]  SumNumOutMin=[]  SumNumOutMax=[]  DivideOutMin=[]  DivideOutMax=[]  UdiffTsProdOutMin=[]  UdiffTsProdOutMax=[]  NTsProdOutMin=[]  NTsProdOutMax=[]  UintegralTsProdOutMin=[]  UintegralTsProdOutMax=[]  UngainTsProdOutMin=[]  UngainTsProdOutMax=[]  ClampingZeroOutDataTypeStr=Inherit: Inherit via back propagation  ClampingZeroOutMin=[]  ClampingZeroOutMax=[]  FilterDenConstantOutDataTypeStr=Inherit: Inherit via back propagation  FilterDenConstantOutMin=[]  FilterDenConstantOutMax=[]  PCopyOutDataTypeStr=Inherit: Inherit via back propagation  PCopyOutMin=[]  PCopyOutMax=[]  NCopyOutDataTypeStr=Inherit: Inherit via back propagation  NCopyOutMin=[]  NCopyOutMax=[]  IntegratorContinuousStateAttributes=''  IntegratorStateMustResolveToSignalObject=off  IntegratorRTWStateStorageClass=Auto  FilterContinuousStateAttributes=''  FilterStateMustResolveToSignalObject=off  FilterRTWStateStorageClass=Auto  ParallelPVariant=InternalParameters  IdealPVariant=Disabled  IVariant=InternalParameters  DVariant=Disabled  IntegratorVariant=Discrete  SatVariant=Disabled  AWVariant=Passthrough  PCopyVariant=Disabled  TRVariant=Disabled  FdbkBlocksVariant=Forward  IdealPFdbkVariant=Disabled  SatFdbkVariant=Disabled  DerivativeFilterVariant=Disabled  NVariant=Disabled  NCopyVariant=Disabled_SignalSpec  FilterICVariant=Disabled  IntegratorICVariant=InternalICs  ExternalResetVariant=Disabled  TRSumVariant=Passthrough  SumFdbkVariant=Disabled  SumVariant=Sum_PI  TsampFilterVariant=InternalTs  TsampNgainVariant=Passthrough  TsampIntegralVariant=Disabled_SignalSpec  ExternalSaturationOutDataTypeStr=Inherit: Same as second input
  PID Controller4 : slpidlib/PID Controller  Controller=PI  Form=Parallel  TimeDomain=Discrete-time  UseExternalTs=off  SampleTime=-1  IntegratorMethod=Forward Euler  FilterMethod=Forward Euler  ControllerParametersSource=internal  P=P  I=I  UseKiTs=off  D=30  N=100  UseFilter=on  TunerSelectOption=Transfer Function Based (PID Tuner App)  InitialConditionSource=internal  InitialConditionForIntegrator=0  InitialConditionForFilter=0  DifferentiatorICPrevScaledInput=0  ExternalReset=none  TrackingMode=off  Kt=1  LimitOutput=off  SatLimitsSource=internal  UpperSaturationLimit=inf  LowerSaturationLimit=-inf  LinearizeAsGain=on  AntiWindupMode=none  Kb=1  LimitIntegrator=off  UpperIntegratorSaturationLimit=inf  LowerIntegratorSaturationLimit=-inf  POutMin=[]  POutMax=[]  IOutMin=[]  IOutMax=[]  DOutMin=[]  DOutMax=[]  NOutMin=[]  NOutMax=[]  SumOutMin=[]  SumOutMax=[]  SaturationOutMin=[]  SaturationOutMax=[]  PParamMin=[]  PParamMax=[]  IParamMin=[]  IParamMax=[]  DParamMin=[]  DParamMax=[]  NParamMin=[]  NParamMax=[]  KbParamMin=[]  KbParamMax=[]  KtParamMin=[]  KtParamMax=[]  KbOutMin=[]  KbOutMax=[]  KtOutMin=[]  KtOutMax=[]  IntegratorOutMin=[]  IntegratorOutMax=[]  FilterOutMin=[]  FilterOutMax=[]  SumI1OutMin=[]  SumI1OutMax=[]  SumI2OutMin=[]  SumI2OutMax=[]  SumI3OutMin=[]  SumI3OutMax=[]  SumI4OutMin=[]  SumI4OutMax=[]  SumDOutMin=[]  SumDOutMax=[]  DifferentiatorOutMin=[]  DifferentiatorOutMax=[]  FilterDiffOutCoefMin=[]  FilterDiffOutCoefMax=[]  ReciprocalOutMin=[]  ReciprocalOutMax=[]  SumDenOutMin=[]  SumDenOutMax=[]  SumNumOutMin=[]  SumNumOutMax=[]  DivideOutMin=[]  DivideOutMax=[]  UdiffTsProdOutMin=[]  UdiffTsProdOutMax=[]  NTsProdOutMin=[]  NTsProdOutMax=[]  UintegralTsProdOutMin=[]  UintegralTsProdOutMax=[]  UngainTsProdOutMin=[]  UngainTsProdOutMax=[]  ClampingZeroOutDataTypeStr=Inherit: Inherit via back propagation  ClampingZeroOutMin=[]  ClampingZeroOutMax=[]  FilterDenConstantOutDataTypeStr=Inherit: Inherit via back propagation  FilterDenConstantOutMin=[]  FilterDenConstantOutMax=[]  PCopyOutDataTypeStr=Inherit: Inherit via back propagation  PCopyOutMin=[]  PCopyOutMax=[]  NCopyOutDataTypeStr=Inherit: Inherit via back propagation  NCopyOutMin=[]  NCopyOutMax=[]  IntegratorContinuousStateAttributes=''  IntegratorStateMustResolveToSignalObject=off  IntegratorRTWStateStorageClass=Auto  FilterContinuousStateAttributes=''  FilterStateMustResolveToSignalObject=off  FilterRTWStateStorageClass=Auto  ParallelPVariant=InternalParameters  IdealPVariant=Disabled  IVariant=InternalParameters  DVariant=Disabled  IntegratorVariant=Discrete  SatVariant=Disabled  AWVariant=Passthrough  PCopyVariant=Disabled  TRVariant=Disabled  FdbkBlocksVariant=Forward  IdealPFdbkVariant=Disabled  SatFdbkVariant=Disabled  DerivativeFilterVariant=Disabled  NVariant=Disabled  NCopyVariant=Disabled_SignalSpec  FilterICVariant=Disabled  IntegratorICVariant=InternalICs  ExternalResetVariant=Disabled  TRSumVariant=Passthrough  SumFdbkVariant=Disabled  SumVariant=Sum_PI  TsampFilterVariant=InternalTs  TsampNgainVariant=Passthrough  TsampIntegralVariant=Disabled_SignalSpec  ExternalSaturationOutDataTypeStr=Inherit: Same as second input
  PWM Generator (2-Level)1 : spsPWMGenerator2LevelLib/PWM Generator (2-Level)  ModulatorType=Three-phase bridge (6 pulses)  ModulatorMode=Unsynchronized  Fc=10e3  Pc=0  nF=27  MinMax="[ -1  1 ]"  SamplingTechnique=Natural  ModulatingSignals=off  m=0.8  Freq=60  Phase=0  Ts=0  ShowCarrierOutport=off
  Product{1..4} (4 alike) : Product
  Scope : Scope  NumInputPorts=2
  Sum : Sum  Inputs=-+|
  Sum1 : Sum  Inputs=|+-
  Sum2 : Sum  Inputs=|+-
  Sum3 : Sum  Inputs=|+-
  Sum4 : Sum  Inputs=++-
  Sum5 : Sum  Inputs=++|
  Sum6 : Sum  Inputs=-+|
  Sum7 : Sum  Inputs=+++
  dq0 to abc1 : spsdq0toabcLib/dq0 to abc  Alignment=90 degrees behind phase A axis
  wC : Subsystem
  wL : Subsystem
  PWM : Outport
  tag scope: Uref_1=global
  wires:
  Mux2/1 -> Scope/2
  Mux1/1 -> Scope/1
  Vqref/1 -> Sum2/1, Mux2/1
  Vdref/1 -> Sum/2, Mux1/1
  Sum5/1 -> Sum6/2
  Sum1/1 -> Sum3/1
  Product1/1 -> Sum1/2
  wC/1(wC) -> Product1/1, Product2/2
  Sum/1 -> PID Controller1/1
  Product2/1 -> Sum5/1
  Constant2/1 -> wC/1(f)
  PID Controller1/1 -> Sum1/1
  Vq/1 -> Sum2/2, Sum7/3, Product1/2, Mux2/2
  Vd/1 -> Product2/1, Sum4/1, Mux1/2, Sum/1
  PID Controller4/1 -> Sum5/2
  Sum2/1 -> PID Controller4/1
  ILq/1 -> Sum6/1, Product3/2
  Sum7/1 -> Mux/2
  Sum4/1 -> Mux/1
  Constant1/1 -> wL/1(f)
  dq0 to abc1/1 -> PWM Generator (2-Level)1/1, [Uref_1]
  Mux/1 -> dq0 to abc1/1
  PWM Generator (2-Level)1/1 -> PWM/1
  PID Controller/1 -> Sum4/2
  Sum3/1 -> PID Controller/1
  Product3/1 -> Sum4/3
  Product4/1 -> Sum7/1
  PID Controller2/1 -> Sum7/2
  Sum6/1 -> PID Controller2/1
  wL/1(wL) -> Product3/1, Product4/2
  ILd/1 -> Product4/1, Sum3/2
  Constant/1 -> Mux/3
  [wt_1] -> dq0 to abc1/2

== system supplemental_network/VSG_1/ 调制/Subsystem/电压电流双闭环/wC ==
  f : Inport
  Gain : Gain  Gain=2*pi*Cf*SB/(UB^2)
  wC : Outport
  wires:
  Gain/1 -> wC/1
  f/1 -> Gain/1

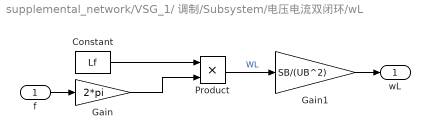
== system supplemental_network/VSG_1/ 调制/Subsystem/电压电流双闭环/wL ==
  f : Inport
  Constant : Constant  Value=Lf
  Gain : Gain  Gain=2*pi
  Gain1 : Gain  Gain=SB/(UB^2)
  Product : Product
  wL : Outport
  wires:
  Gain1/1 -> wL/1
  f/1 -> Gain/1
  Constant/1 -> Product/1
  Product/1 -> Gain1/1  "WL"
  Gain/1 -> Product/2

== matlab function supplemental_network/Aggregate renewable injection ==
  data: v input; ia output; t input; enabled input; ib output; ic output; P output
function [ia,ib,ic,P]=renewable(v,t,enabled)
P=0;
if enabled>0.5 && t>=1
P=3000*(1+0.5*sin(2*pi*2*(t-1)));
end
den=max(sum(v.^2),1e4);
i=-P*v/den;
ia=i(1);ib=i(2);ic=i(3);
end

== matlab function supplemental_network/可编程电源/Embedded MATLAB Function ==
  data: t input; fs input; Kt input; Ua output; U1 input; U5 input; Ub output; Uc output; U7 input; ena output
function [Ua,Ub,Uc,ena] = fcn(t,fs,Kt,U1,U5,U7)
% This block supports the Embedded MATLAB subset.
% See the help menu for details. 

if(t<Kt)
    Ua=U1*sin(2*pi*fs*t);
    Ub=U1*sin(2*pi*fs*t-2*pi/3);
    Uc=U1*sin(2*pi*fs*t+2*pi/3);
    ena=0;
else
    Ua=U1*sin(2*pi*fs*t)+U5*sin(2*pi*fs*5*t)+U7*sin(2*pi*fs*7*t);
    Ub=U1*sin(2*pi*fs*t-2*pi/3)+U5*sin(2*pi*fs*5*t-2*pi/3)+U7*sin(2*pi*fs*7*t-2*pi/3);
    Uc=U1*sin(2*pi*fs*t+2*pi/3)+U5*sin(2*pi*fs*5*t+2*pi/3)+U7*sin(2*pi*fs*7*t+2*pi/3);
    ena=1;
end
